simulink model "transmisor"  (R2026a)
settings: Solver=FixedStepAuto  StopTime=Tsim  FixedStep=Ts
InitFcn:
  | tx_params
values from neighbouring files (symbols this model uses):
  K_FDM = 1/3    (= 0.333333333333)    [tx_params.m]
  Ts = 1/Fs    (= 2e-07)    [tx_params.m]
libraries: commanapbnd3 x4
settings Model: Creator=felipe  LastModifiedBy=felipe

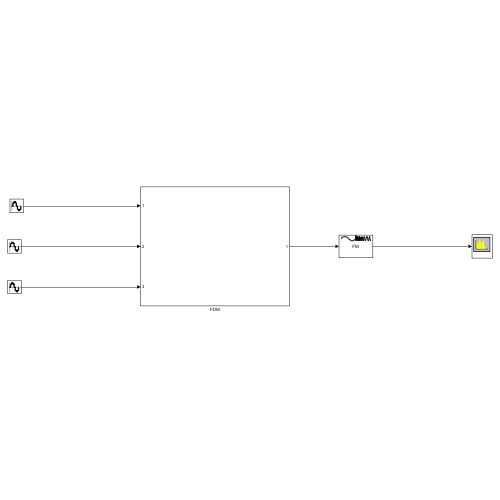
[thumbnail: Simulink's stored preview of the top-level diagram]
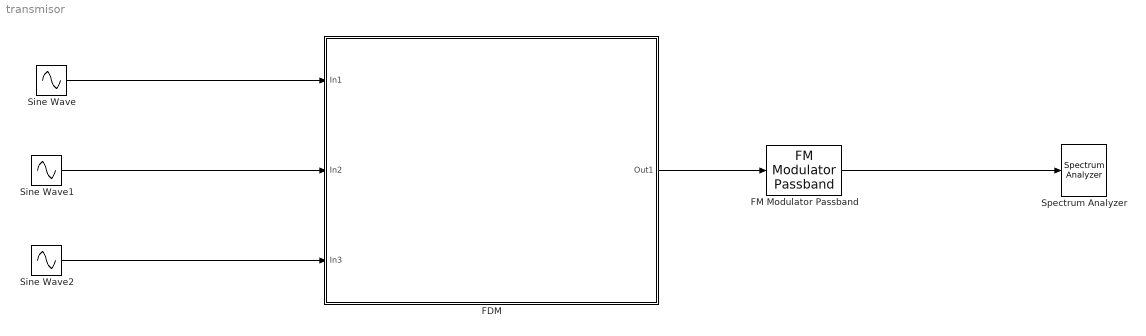
== system transmisor ==
  FDM : Subsystem
  FM Modulator Passband : commanapbnd3/FM Modulator Passband  Fc=fc_tx  Ph=0  Kc=deltaf
  Sine Wave : Sin  Frequency=2*pi*1000  SampleTime=Ts
  Sine Wave1 : Sin  Frequency=2*pi*3000  SampleTime=Ts
  Sine Wave2 : Sin  Frequency=2*pi*6000  SampleTime=Ts
  Spectrum Analyzer : SpectrumAnalyzer  WindowPosition=[394.000000,230.000000,800.000000,500.000000,]  Visible=on  ScopeFrameLocation=window  SpectrumType=Power density  Method=Welch  PlotAsTwoSidedSpectrum=off  RBWSource=Property  RBW=1e3  FrequencySpan=Start and stop frequencies  Span=100e3  CenterFrequency=2e6  StartFrequency=1.8e6  StopFrequency=2.2e6  AveragingMethod=Exponential  SpectrumUnits=dBm/Hz  YLimits=[-228.9707 54.2512]
  wires:
  FDM/1(Out1) -> FM Modulator Passband/1
  Sine Wave2/1 -> FDM/3(In3)
  Sine Wave/1 -> FDM/1(In1)
  Sine Wave1/1 -> FDM/2(In2)
  FM Modulator Passband/1 -> Spectrum Analyzer/1

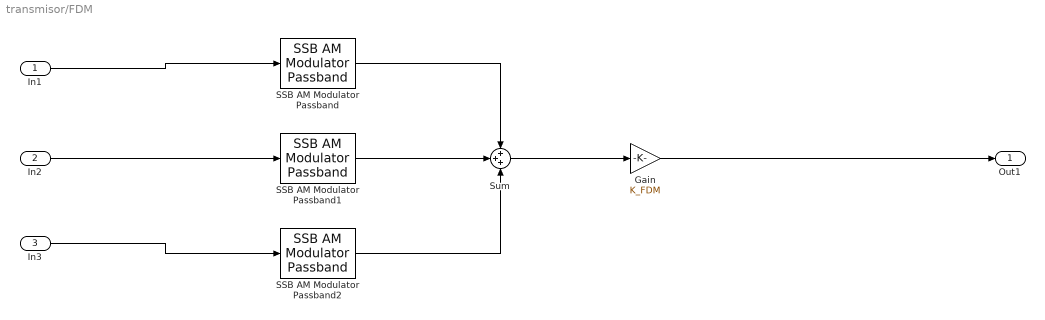
== system transmisor/FDM ==
  In1 : Inport
  In2 : Inport  Port=2
  In3 : Inport  Port=3
  Gain : Gain  Gain=K_FDM
  SSB AM Modulator Passband : commanapbnd3/SSB AM Modulator Passband  Fc=fc1  Ph=0  Sd=Upper  Ho=Nh
  SSB AM Modulator Passband1 : commanapbnd3/SSB AM Modulator Passband  Fc=fc2  Ph=0  Sd=Upper  Ho=Nh
  SSB AM Modulator Passband2 : commanapbnd3/SSB AM Modulator Passband  Fc=fc3  Ph=0  Sd=Upper  Ho=Nh
  Sum : Sum  Inputs=+++
  Out1 : Outport
  wires:
  SSB AM Modulator Passband1/1 -> Sum/2
  SSB AM Modulator Passband2/1 -> Sum/3
  Sum/1 -> Gain/1
  SSB AM Modulator Passband/1 -> Sum/1
  Gain/1 -> Out1/1
  In3/1 -> SSB AM Modulator Passband2/1
  In2/1 -> SSB AM Modulator Passband1/1
  In1/1 -> SSB AM Modulator Passband/1
